simulink model "structure_body6dof"  (R2026b)
settings: Solver=VariableStepAuto
undefined symbols (not defined in the file or in its folder): P
libraries: aerolib6dof2 x2, sharedutil x2
settings Model: Creator=aomar  LastModifiedBy=aomar

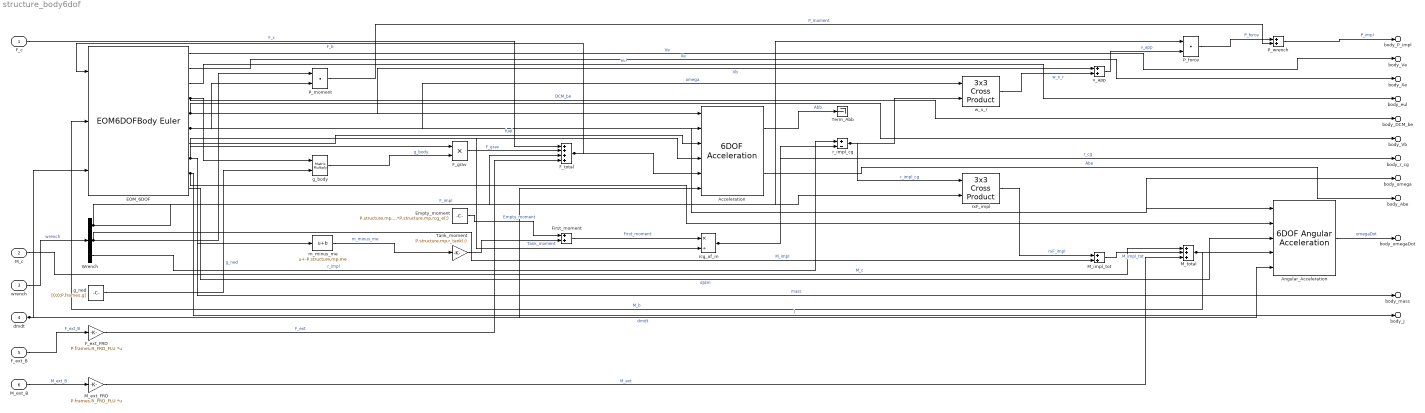
== system structure_body6dof ==
  F_c : Inport
  M_c : Inport  Port=2
  wrench : Inport  Port=3
  dmdt : Inport  Port=4
  F_ext_B : Inport  Port=5
  M_ext_B : Inport  Port=6
  Acceleration : aerolib6dof2/6DOF Acceleration  units=Metric (MKS)  mtype=Simple Variable  vre_flag=off
  Angular_Acceleration : aerolib6dof2/6DOF Angular Acceleration  units=Metric (MKS)  mtype=Simple Variable
  EOM_6DOF : EOM6DOFBodyEuler  mtype=Simple Variable  xme_0=P.structure.init.xme0  Vm_0=P.structure.init.Vb0  eul_0=P.structure.init.eul0  mass_0=P.structure.mp.m0  mass_e=P.structure.mp.me  mass_f=P.structure.mp.mf  inertia_e=P.structure.mp.Je  inertia_f=P.structure.mp.Jf  mass_flag=on  zeroCrossing=off
  Empty_moment : Constant  Value=P.structure.mp.me*P.structure.mp.rcg_e(:)  VectorParams1D=off
  F_ext_FRD : Gain  Gain=P.frames.R_FRD_FLU  Multiplication=Matrix(K*u)
  F_grav : Product  Inputs=**
  F_total : Sum  Inputs=++++
  First_moment : Sum
  M_ext_FRD : Gain  Gain=P.frames.R_FRD_FLU  Multiplication=Matrix(K*u)
  M_impl_tot : Sum
  M_total : Sum  Inputs=+++
  P_force : DotProduct  OutDataTypeStr=Inherit: Inherit via internal rule
  P_moment : DotProduct  OutDataTypeStr=Inherit: Inherit via internal rule
  P_wrench : Sum
  Tank_moment : Gain  Gain=P.structure.mp.r_tank(:)
  Term_Abb : Terminator
  Wrench : Demux  Outputs=[3 3 3]
  g_body : Product  Inputs=**  Multiplication=Matrix(*)
  g_ned : Constant  Value=[0;0;P.frames.g]  VectorParams1D=off
  m_minus_me : Bias  Bias=-P.structure.mp.me  SaturateOnIntegerOverflow=off
  r_impl_cg : Sum  Inputs=+-
  rcg_of_m : Product  Inputs=*/
  rxF_impl : sharedutil/3x3 Cross Product  aMode=aMode
      settings: LibrarySourceBlock=aerolibutil/3x3 Cross Product
  v_app : Sum
  w_x_r : sharedutil/3x3 Cross Product  aMode=aMode
      settings: LibrarySourceBlock=aerolibutil/3x3 Cross Product
  body_Xe : Outport  PortName=body  Element=Xe
  body_Ve : Outport  PortName=body  Element=Ve
  body_eul : Outport  PortName=body  Element=eul
  body_DCM_be : Outport  PortName=body  Element=DCM_be
  body_Vb : Outport  PortName=body  Element=Vb
  body_omega : Outport  PortName=body  Element=omega
  body_mass : Outport  PortName=body  Element=mass
  body_J : Outport  PortName=body  Element=J
  body_Abe : Outport  PortName=body  Element=Abe
  body_omegaDot : Outport  PortName=body  Element=omegaDot
  body_r_cg : Outport  PortName=body  Element=r_cg
  body_P_impl : Outport  PortName=body  Element=P_impl
  wires:
  F_c/1 -> F_total/1  "F_c"
  M_c/1 -> M_total/1  "M_c"
  wrench/1 -> Wrench/1  "wrench"
  dmdt/1 -> EOM_6DOF/3, Acceleration/6, Angular_Acceleration/5  "dmdt"
  F_ext_B/1 -> F_ext_FRD/1  "F_ext_B"
  M_ext_B/1 -> M_ext_FRD/1  "M_ext_B"
  Wrench/1 -> P_force/1, F_total/3, rxF_impl/2  "F_impl"
  Wrench/2 -> P_moment/1, M_impl_tot/2  "M_impl"
  Wrench/3 -> r_impl_cg/1  "r_impl"
  g_ned/1 -> g_body/2  "g_ned"
  F_ext_FRD/1 -> F_total/4  "F_ext"
  M_ext_FRD/1 -> M_total/3  "M_ext"
  EOM_6DOF/1 -> body_Ve/1  "Ve"
  EOM_6DOF/2 -> body_Xe/1  "Xe"
  EOM_6DOF/3 -> body_eul/1  "eul"
  EOM_6DOF/4 -> g_body/1, body_DCM_be/1  "DCM_be"
  EOM_6DOF/5 -> v_app/1, body_Vb/1, Acceleration/1  "Vb"
  EOM_6DOF/7 -> Acceleration/3  "fuel"
  EOM_6DOF/10 -> Angular_Acceleration/3  "dJdm"
  P_moment/1 -> P_wrench/2  "P_moment"
  g_body/1 -> F_grav/2  "g_body"
  m_minus_me/1 -> Tank_moment/1  "m_minus_me"
  F_grav/1 -> F_total/2  "F_grav"
  Empty_moment/1 -> First_moment/1  "Empty_moment"
  Tank_moment/1 -> First_moment/2  "Tank_moment"
  F_total/1 -> EOM_6DOF/1, Acceleration/5  "F_b"
  First_moment/1 -> rcg_of_m/1  "First_moment"
  rcg_of_m/1 -> r_impl_cg/2, body_r_cg/1  "r_cg"
  Acceleration/1 -> Term_Abb/1  "Abb"
  Acceleration/2 -> body_Abe/1  "Abe"
  r_impl_cg/1 -> w_x_r/2, rxF_impl/1  "r_impl_cg"
  w_x_r/1 -> v_app/2  "w_x_r"
  rxF_impl/1 -> M_impl_tot/1  "rxF_impl"
  v_app/1 -> P_force/2  "v_app"
  M_impl_tot/1 -> M_total/2  "M_impl_tot"
  M_total/1 -> EOM_6DOF/2, Angular_Acceleration/4  "M_b"
  P_force/1 -> P_wrench/1  "P_force"
  P_wrench/1 -> body_P_impl/1  "P_impl"
  Angular_Acceleration/1 -> body_omegaDot/1  "omegaDot"
  EOM_6DOF/6 -> Angular_Acceleration/1, body_omega/1, P_moment/2, w_x_r/1, Acceleration/2  "omega"
  EOM_6DOF/8 -> body_mass/1, rcg_of_m/2, m_minus_me/1, F_grav/1, Acceleration/4  "mass"
  EOM_6DOF/9 -> body_J/1, Angular_Acceleration/2  "J"
